simulink model "PV_WIND_BESS_ISLAND_R1"  (R2023b)
settings: Solver=ode14x  StartTime=0.0  StopTime=3.2  FixedStep=25e-6  MaxStep=1e-5  RelTol=1e-3
InitFcn:
  | setup_v2_paths;init_grid_supported_integration;run(which('init_bess_vsm_r10.m'));
undefined symbols (not defined in the file): Base, Control, Converter, DiscIntNeverNeededParam, Drive, Filter, G, PMSG, V2, Wind
libraries: nesl_utility x51, ee_lib x44, fl_lib x25, simulink x6
(part 2 of 4)

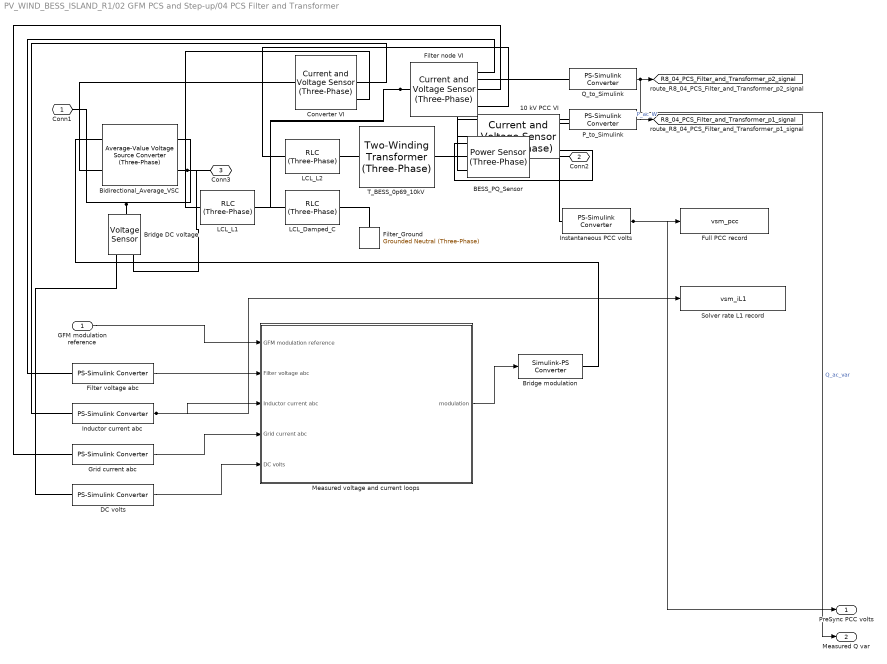
== system PV_WIND_BESS_ISLAND_R1/02 GFM PCS and Step-up/04 PCS Filter and Transformer ==
  GFM modulation reference : Inport
  10 kV PCC VI : ee_lib/Sensors & Transducers/Current and Voltage Sensor (Three-Phase)  port_option=ee.enum.threePhasePort.composite  vMeasurementType=ee.enum.vmeasurement.lg  outputUnit=ee.enum.unit.si  SRated=100e6 A*V  VRated=24e3 V  I_specify=off  I_priority=None  I=[0, 0, 0] A  I_nominal_specify=off  I_nominal_value=1  I_nominal_unit=A  V_specify=off  V_priority=None  V=[0, 0, 0] V  V_nominal_specify=off  V_nominal_value=1  V_nominal_unit=V
  BESS_PQ_Sensor : ee_lib/Sensors & Transducers/Power Sensor (Three-Phase)  port_option=ee.enum.threePhasePort.composite  load_type=ee.enum.passive.type_balanced.balanced  f0=60 Hz
  Bidirectional_Average_VSC : ee_lib/Semiconductors & Converters/Converters/Average-Value Voltage Source Converter (Three-Phase)  port_option=ee.enum.threePhasePort.composite  enable_block_pulses_input=false  krec=G.dc.Rbattery_ohm/10 Ohm  frequency_option=ee.enum.converters.frequency.variable  input_option=ee.enum.converters.inputOption.ModWave  FRated=G.f0_Hz Hz  losses_parameterization=ee.enum.converters.losses.fixed  Pfixed=1 W  ks=0.01  kc1=1.7 V  kc2=0.01 Ohm  Ploss_vect=[100, 800, 1870, 3250, 4900] W  Irms_vect=[10, 100, 200, 300, 400] A  Vdc_nom=300 V  thermal_mass=30000 J/K  temperature_specify=off  temperature_priority=High  temperature=298.15 K  temperature_nominal_specify=off  temperature_nominal_value=1  temperature_nominal_unit=K
  Bridge DC voltage : fl_lib/Electrical/Electrical Sensors/Voltage Sensor
  Bridge modulation : nesl_utility/Simulink-PS Converter  PhysicalDomain=network_engine_domain  SubClassName=ps_input  LeftPortType=input  RightPortType=output  PseudoPeriodic=off  Frequencies=[]  NoiseDistribution=none  NoiseParameters=[]  Unit=1  AffineConversion=off  FilteringAndDerivatives=zero  SimscapeFilterOrder=1  InputFilterTimeConstant=0.001  UdotUserProvided=0
  Converter VI : ee_lib/Sensors & Transducers/Current and Voltage Sensor (Three-Phase)  port_option=ee.enum.threePhasePort.composite  vMeasurementType=ee.enum.vmeasurement.lg  outputUnit=ee.enum.unit.si  SRated=100e6 A*V  VRated=24e3 V  I_specify=off  I_priority=None  I=[0, 0, 0] A  I_nominal_specify=off  I_nominal_value=1  I_nominal_unit=A  V_specify=off  V_priority=None  V=[0, 0, 0] V  V_nominal_specify=off  V_nominal_value=1  V_nominal_unit=V
  DC volts : nesl_utility/PS-Simulink Converter  PhysicalDomain=network_engine_domain  SubClassName=ps_output  LeftPortType=input  RightPortType=output  PseudoPeriodic=off  Frequencies=[]  VectorFormat=inherit  Unit=V  AffineConversion=off
  Filter node VI : ee_lib/Sensors & Transducers/Current and Voltage Sensor (Three-Phase)  port_option=ee.enum.threePhasePort.composite  vMeasurementType=ee.enum.vmeasurement.lg  outputUnit=ee.enum.unit.si  SRated=100e6 A*V  VRated=24e3 V  I_specify=off  I_priority=None  I=[0, 0, 0] A  I_nominal_specify=off  I_nominal_value=1  I_nominal_unit=A  V_specify=off  V_priority=None  V=[0, 0, 0] V  V_nominal_specify=off  V_nominal_value=1  V_nominal_unit=V
  Filter voltage abc : nesl_utility/PS-Simulink Converter  PhysicalDomain=network_engine_domain  SubClassName=ps_output  LeftPortType=input  RightPortType=output  PseudoPeriodic=off  Frequencies=[]  VectorFormat=inherit  Unit=V  AffineConversion=off
  Filter_Ground : ee_lib/Connectors & References/Grounded Neutral (Three-Phase)  port_option=ee.enum.threePhasePort.composite
  Full PCC record : ToWorkspace  VariableName=vsm_pcc  SaveFormat=Timeseries  SampleTime=-1
  Grid current abc : nesl_utility/PS-Simulink Converter  PhysicalDomain=network_engine_domain  SubClassName=ps_output  LeftPortType=input  RightPortType=output  PseudoPeriodic=off  Frequencies=[]  VectorFormat=inherit  Unit=A  AffineConversion=off
  Inductor current abc : nesl_utility/PS-Simulink Converter  PhysicalDomain=network_engine_domain  SubClassName=ps_output  LeftPortType=input  RightPortType=output  PseudoPeriodic=off  Frequencies=[]  VectorFormat=inherit  Unit=A  AffineConversion=off
  Instantaneous PCC volts : nesl_utility/PS-Simulink Converter  PhysicalDomain=network_engine_domain  SubClassName=ps_output  LeftPortType=input  RightPortType=output  PseudoPeriodic=off  Frequencies=[]  VectorFormat=inherit  Unit=V  AffineConversion=off
  LCL_Damped_C : ee_lib/Passive/RLC Assemblies/RLC (Three-Phase)  port_option=ee.enum.threePhasePort.composite  component_structure=ee.enum.rlc.structure.SeriesRC  R=G.filter.Rd_ohm Ohm  L=1e-3 H  C=G.filter.C_F F  R_parasitic=0 Ohm  G_parasitic=0 1/Ohm  IL_specify=off  IL_priority=High  IL=[0, 0, 0] A  IL_nominal_specify=off  IL_nominal_value=1  IL_nominal_unit=A  VC_specify=off  VC_priority=High  VC=[0, 0, 0] V  VC_nominal_specify=off  VC_nominal_value=1  VC_nominal_unit=V
  LCL_L1 : ee_lib/Passive/RLC Assemblies/RLC (Three-Phase)  port_option=ee.enum.threePhasePort.composite  component_structure=ee.enum.rlc.structure.SeriesRL  R=G.filter.R1_ohm Ohm  L=G.filter.L1_H H  C=1e-6 F  R_parasitic=0 Ohm  G_parasitic=0 1/Ohm  IL_specify=off  IL_priority=High  IL=[0, 0, 0] A  IL_nominal_specify=off  IL_nominal_value=1  IL_nominal_unit=A  VC_specify=off  VC_priority=High  VC=[0, 0, 0] V  VC_nominal_specify=off  VC_nominal_value=1  VC_nominal_unit=V
  LCL_L2 : ee_lib/Passive/RLC Assemblies/RLC (Three-Phase)  port_option=ee.enum.threePhasePort.composite  component_structure=ee.enum.rlc.structure.SeriesRL  R=G.filter.R2_ohm Ohm  L=G.filter.L2_H H  C=1e-6 F  R_parasitic=0 Ohm  G_parasitic=0 1/Ohm  IL_specify=off  IL_priority=High  IL=[0, 0, 0] A  IL_nominal_specify=off  IL_nominal_value=1  IL_nominal_unit=A  VC_specify=off  VC_priority=High  VC=[0, 0, 0] V  VC_nominal_specify=off  VC_nominal_value=1  VC_nominal_unit=V
  Measured voltage and current loops : Subsystem
  P_to_Simulink : nesl_utility/PS-Simulink Converter  PhysicalDomain=network_engine_domain  SubClassName=ps_output  LeftPortType=input  RightPortType=output  PseudoPeriodic=off  Frequencies=[]  VectorFormat=inherit  Unit=W  AffineConversion=off
  Q_to_Simulink : nesl_utility/PS-Simulink Converter  PhysicalDomain=network_engine_domain  SubClassName=ps_output  LeftPortType=input  RightPortType=output  PseudoPeriodic=off  Frequencies=[]  VectorFormat=inherit  Unit=W  AffineConversion=off
  Solver rate L1 record : ToWorkspace  VariableName=vsm_iL1  SaveFormat=Timeseries  SampleTime=-1
  T_BESS_0p69_10kV : ee_lib/Passive/Transformers/Two-Winding Transformer (Three-Phase)  SRated=G.transformer.S_VA A*V  FRated=G.f0_Hz Hz  Winding1Connection=ee.enum.windingconnection.delta1  VRated1=G.ac.Vll_low_V V  Winding2Connection=ee.enum.windingconnection.Yg  VRated2=G.ac.Vll_high_V V  CoreType=ee.enum.coretype.threelimb  pu_Rw1=G.transformer.pu_Rw1  pu_Rw2=G.transformer.pu_Rw2  leakage_reactance_option=ee.enum.transformer_leakage.include  pu_Xl1=G.transformer.pu_Xl1  pu_Xl2=G.transformer.pu_Xl2  magnetizing_resistance_option=ee.enum.transformer_magnetizingResistance.exclude  pu_Rm=500  magnetizing_reactance_option=ee.enum.transformer_magnetizingReactance.exclude  saturation_option=ee.enum.transformer_saturation.exclude  pu_Xm=500  current_data=[0, .002, 1, 2]  magnetic_flux_data=[0, 1.2, 1.5, 1.51]  pu_X0=0.5  i1_specify=off  i1_priority=None  i1=[0, 0, 0] A  i1_nominal_specify=off  i1_nominal_value=1  i1_nominal_unit=A  i2_specify=off  i2_priority=None  i2=[0, 0, 0] A  i2_nominal_specify=off  i2_nominal_value=1  i2_nominal_unit=A  phi_specify=off  phi_priority=None  phi=[0, 0, 0]  phi_nominal_specify=off  phi_nominal_value=1  phi_nominal_unit=1
  Conn1 : PMIOPort  Side=Right  ConnectionType=Connection: foundation.electrical.electrical
  Conn2 : PMIOPort  Port=2  Side=Right  ConnectionType=Connection: foundation.electrical.three_phase
  Conn3 : PMIOPort  Port=3  Side=Right  ConnectionType=Connection: foundation.electrical.electrical
  PreSync PCC volts : Outport
  Measured Q var : Outport  Port=2
  tag scope: R8_04_PCS_Filter_and_Transformer_p1_signal=global, R8_04_PCS_Filter_and_Transformer_p2_signal=global
  wires:
  P_to_Simulink/1 -> [R8_04_PCS_Filter_and_Transformer_p1_signal]  "P_ac_W"
  Q_to_Simulink/1 -> [R8_04_PCS_Filter_and_Transformer_p2_signal], Measured Q var/1  "Q_ac_var"
  GFM modulation reference/1 -> Measured voltage and current loops/1(GFM modulation reference)
  Filter voltage abc/1 -> Measured voltage and current loops/2(Filter voltage abc)
  Inductor current abc/1 -> Measured voltage and current loops/3(Inductor current abc), Solver rate L1 record/1
  Grid current abc/1 -> Measured voltage and current loops/4(Grid current abc)
  DC volts/1 -> Measured voltage and current loops/5(DC volts)
  Measured voltage and current loops/1(modulation) -> Bridge modulation/1
  Instantaneous PCC volts/1 -> Full PCC record/1, PreSync PCC volts/1
  connections:
  BESS_PQ_Sensor/RConn1 -- Conn2/RConn1
  BESS_PQ_Sensor/LConn3 -- Q_to_Simulink/LConn1
  LCL_Damped_C/RConn1 -- Filter_Ground/LConn1
  LCL_L2/RConn1 -- T_BESS_0p69_10kV/LConn1
  Conn3/RConn1 -- Bidirectional_Average_VSC/RConn2 -- Bridge DC voltage/RConn2
  BESS_PQ_Sensor/LConn2 -- P_to_Simulink/LConn1
  Bidirectional_Average_VSC/RConn1 -- Conn1/RConn1 -- Bridge DC voltage/LConn1
  Bidirectional_Average_VSC/LConn2 -- Converter VI/LConn1
  Converter VI/RConn3 -- LCL_L1/LConn1
  LCL_Damped_C/LConn1 -- LCL_L1/RConn1 -- Filter node VI/LConn1
  Filter node VI/RConn3 -- LCL_L2/LConn1
  Filter node VI/RConn1 -- Filter voltage abc/LConn1
  Converter VI/RConn2 -- Inductor current abc/LConn1
  Filter node VI/RConn2 -- Grid current abc/LConn1
  Bridge DC voltage/RConn1 -- DC volts/LConn1
  Bridge modulation/RConn1 -- Bidirectional_Average_VSC/LConn1
  T_BESS_0p69_10kV/RConn1 -- 10 kV PCC VI/LConn1
  10 kV PCC VI/RConn3 -- BESS_PQ_Sensor/LConn1
  10 kV PCC VI/RConn1 -- Instantaneous PCC volts/LConn1

== system PV_WIND_BESS_ISLAND_R1/PV Resource/01 PV Array ==
  Array VI : Mux  Inputs=2
  Current SI : nesl_utility/PS-Simulink Converter  PhysicalDomain=network_engine_domain  SubClassName=ps_output  LeftPortType=input  RightPortType=output  PseudoPeriodic=off  Frequencies=[]  VectorFormat=inherit  Unit=A  AffineConversion=off
  Irradiance : Constant  Value=V2.PV.dynamic.irradiance_Wpm2
  Irradiance PS : nesl_utility/Simulink-PS Converter  PhysicalDomain=network_engine_domain  SubClassName=ps_input  LeftPortType=input  RightPortType=output  PseudoPeriodic=off  Frequencies=[]  NoiseDistribution=none  NoiseParameters=[]  Unit=W/m^2  AffineConversion=off  FilteringAndDerivatives=zero  SimscapeFilterOrder=1  InputFilterTimeConstant=0.001  UdotUserProvided=0
  PV Array : ee_lib/Sources/Solar Cell  prm=1  Isc=V2.PV.dynamic.Isc_cell_A A  Voc=V2.PV.dynamic.Voc_cell_V V  Is=1e-6 A  Is2=0 A  Iph=7.34 A  Ir0=1000 W/m^2  ec=1.5  N2=2  Rs=0 Ohm  Rp=inf Ohm  N_series=V2.PV.dynamic.Nseries  N_parallel=V2.PV.dynamic.Nparallel  TIPH1=0 1/K  EG=1.11 eV  TXIS1=3  TXIS2=3  TRS1=0  TRP1=0  Tmeas=25 degC  TFIXED=V2.PV.dynamic.temperature_degC degC  thermal_mass=100 J/K  initial_temperature=25 degC
  PV Current : fl_lib/Electrical/Electrical Sensors/Current Sensor
  PV Input Capacitor : fl_lib/Electrical/Electrical Elements/Capacitor  c=V2.PV.dynamic.Cpv_F F  r=1e-6 Ohm  g=0 1/Ohm  i_specify=off  i_priority=None  i=0 A  i_nominal_specify=off  i_nominal_value=1  i_nominal_unit=A  v_specify=off  v_priority=None  v=0 V  v_nominal_specify=off  v_nominal_value=1  v_nominal_unit=V  vc_specify=on  vc_priority=High  vc=V2.PV.dynamic.Vmp_initial_V V  vc_nominal_specify=off  vc_nominal_value=1  vc_nominal_unit=V
  PV Voltage : fl_lib/Electrical/Electrical Sensors/Voltage Sensor
  Voltage SI : nesl_utility/PS-Simulink Converter  PhysicalDomain=network_engine_domain  SubClassName=ps_output  LeftPortType=input  RightPortType=output  PseudoPeriodic=off  Frequencies=[]  VectorFormat=inherit  Unit=V  AffineConversion=off
  arrayPlus : PMIOPort  Side=Right  ConnectionType=Connection: foundation.electrical.electrical
  arrayMinus : PMIOPort  Port=2  Side=Right  ConnectionType=Connection: foundation.electrical.electrical
  arrayVI : Outport
  wires:
  Array VI/1 -> arrayVI/1
  Current SI/1 -> Array VI/2
  Voltage SI/1 -> Array VI/1
  Irradiance/1 -> Irradiance PS/1
  connections:
  PV Current/RConn1 -- Current SI/LConn1
  PV Voltage/RConn1 -- Voltage SI/LConn1
  arrayMinus/RConn1 -- PV Input Capacitor/RConn1 -- PV Array/RConn1 -- PV Voltage/RConn2
  arrayPlus/RConn1 -- PV Voltage/LConn1 -- PV Current/RConn2 -- PV Input Capacitor/LConn1
  PV Array/LConn2 -- PV Current/LConn1
  Irradiance PS/RConn1 -- PV Array/LConn1

== system PV_WIND_BESS_ISLAND_R1/PV Resource/02 MPPT Boost and DC Link ==
  dispatch : Inport
  arrayVI : Inport  Port=2
  Array measurements : Demux  Outputs=2
  Average Boost : ee_lib/Semiconductors & Converters/Converters/Boost Converter  port_option=ee.enum.controlport.ps  device_type=ee.enum.converters.switchingdevice.averaged  Vf=0.8 V  Ron=0.001 Ohm  Rds=0.001 Ohm  Goff=1e-5 1/Ohm  Vgt=1 V  Vgt_off=-1 V  Ih=1 A  Vth=6 V  K=0  diode_param=ee.enum.converters.protectiondiode.nodynamics  diode_Vf=0.8 V  diode_Ron=0.001 Ohm  diode_Goff=1e-5 1/Ohm  diode_C=50 nF  diode_iRM=-235 A  diode_iF=300 A  diode_idot=-50 A/us  diode_trr_param=ee.enum.converters.diodetrr.trr_factor  diode_trr_factor=3  diode_trr=15 us  diode_Qrr=1500 s*uA  Lf=V2.PV.dynamic.Lboost_H H  Rl=V2.PV.dynamic.Rboost_ohm Ohm  Cf=1e-6 F  Rf=0.001 Ohm  snubber_type=ee.enum.converters.snubber.exclude  Cs=1e-7 F  Rs=0.1 Ohm  iL_specify=off  iL_priority=High  iL=0 A  iL_nominal_specify=off  iL_nominal_value=1  iL_nominal_unit=A  vc_specify=on  vc_priority=High  vc=V2.PV.dynamic.Vdc_ref_V V  vc_nominal_specify=off  vc_nominal_value=1  vc_nominal_unit=V
  Boost Current Record : ToWorkspace  VariableName=pv_boost_current  SaveFormat=Timeseries  SampleTime=-1
  Boost Current SI : nesl_utility/PS-Simulink Converter  PhysicalDomain=network_engine_domain  SubClassName=ps_output  LeftPortType=input  RightPortType=output  PseudoPeriodic=off  Frequencies=[]  VectorFormat=inherit  Unit=A  AffineConversion=off
  Boost Output Current : fl_lib/Electrical/Electrical Sensors/Current Sensor
  DC Ground : fl_lib/Electrical/Electrical Elements/Electrical Reference
  DC Link Capacitor : fl_lib/Electrical/Electrical Elements/Capacitor  c=V2.PV.dynamic.Cdc_F F  r=1e-6 Ohm  g=0 1/Ohm  i_specify=off  i_priority=None  i=0 A  i_nominal_specify=off  i_nominal_value=1  i_nominal_unit=A  v_specify=off  v_priority=None  v=0 V  v_nominal_specify=off  v_nominal_value=1  v_nominal_unit=V  vc_specify=on  vc_priority=High  vc=V2.PV.dynamic.Vdc_ref_V V  vc_nominal_specify=off  vc_nominal_value=1  vc_nominal_unit=V
  DC Link Voltage : fl_lib/Electrical/Electrical Sensors/Voltage Sensor
  DC Link Voltage SI : nesl_utility/PS-Simulink Converter  PhysicalDomain=network_engine_domain  SubClassName=ps_output  LeftPortType=input  RightPortType=output  PseudoPeriodic=off  Frequencies=[]  VectorFormat=inherit  Unit=V  AffineConversion=off
  Duty PS : nesl_utility/Simulink-PS Converter  PhysicalDomain=network_engine_domain  SubClassName=ps_input  LeftPortType=input  RightPortType=output  PseudoPeriodic=off  Frequencies=[]  NoiseDistribution=none  NoiseParameters=[]  Unit=1  AffineConversion=off  FilteringAndDerivatives=zero  SimscapeFilterOrder=1  InputFilterTimeConstant=0.001  UdotUserProvided=0
  Duty Sample Delay : UnitDelay  SampleTime=100e-6
  MPPT and Curtailment : Subsystem
  Telemetry Mux : Mux  Inputs=6
  arrayPlus : PMIOPort  Side=Left  ConnectionType=Connection: foundation.electrical.electrical
  arrayMinus : PMIOPort  Port=2  Side=Left  ConnectionType=Connection: foundation.electrical.electrical
  linkPlus : PMIOPort  Port=3  Side=Right  ConnectionType=Connection: foundation.electrical.electrical
  linkMinus : PMIOPort  Port=4  Side=Right  ConnectionType=Connection: foundation.electrical.electrical
  sourceData : Outport
  wires:
  Telemetry Mux/1 -> sourceData/1
  MPPT and Curtailment/3(Vpv_target) -> Telemetry Mux/6
  MPPT and Curtailment/2(Vmp) -> Telemetry Mux/5
  Duty Sample Delay/1 -> Duty PS/1
  MPPT and Curtailment/1(Duty) -> Telemetry Mux/4, Duty Sample Delay/1
  dispatch/1 -> MPPT and Curtailment/4(Command)
  DC Link Voltage SI/1 -> Telemetry Mux/3, MPPT and Curtailment/3(Vdc)
  Array measurements/2 -> Telemetry Mux/2, MPPT and Curtailment/2(Ipv)
  Array measurements/1 -> Telemetry Mux/1, MPPT and Curtailment/1(Vpv)
  arrayVI/1 -> Array measurements/1
  Boost Current SI/1 -> Boost Current Record/1
  connections:
  Duty PS/RConn1 -- Average Boost/LConn1
  DC Link Voltage/RConn1 -- DC Link Voltage SI/LConn1
  Boost Output Current/RConn1 -- Boost Current SI/LConn1
  linkMinus/RConn1 -- DC Link Capacitor/RConn1 -- DC Link Voltage/RConn2 -- DC Ground/LConn1 -- Average Boost/RConn2
  linkPlus/RConn1 -- DC Link Capacitor/LConn1 -- DC Link Voltage/LConn1 -- Boost Output Current/RConn2
  Average Boost/RConn1 -- Boost Output Current/LConn1
  arrayMinus/RConn1 -- Average Boost/LConn3
  arrayPlus/RConn1 -- Average Boost/LConn2

== system PV_WIND_BESS_ISLAND_R1/PV Resource/03 Average Grid Converter ==
  modulationABC : Inport
  Average VSC : ee_lib/Semiconductors & Converters/Converters/Average-Value Voltage Source Converter (Three-Phase)  port_option=ee.enum.threePhasePort.composite  enable_block_pulses_input=false  krec=0.01 Ohm  frequency_option=ee.enum.converters.frequency.variable  input_option=ee.enum.converters.inputOption.ModWave  FRated=V2.PV.rating.f_Hz Hz  losses_parameterization=ee.enum.converters.losses.fixed  Pfixed=1 W  ks=0.01  kc1=1.7 V  kc2=0.01 Ohm  Ploss_vect=[100, 800, 1870, 3250, 4900] W  Irms_vect=[10, 100, 200, 300, 400] A  Vdc_nom=V2.PV.dynamic.Vdc_ref_V V  thermal_mass=30000 J/K  temperature_specify=off  temperature_priority=High  temperature=298.15 K  temperature_nominal_specify=off  temperature_nominal_value=1  temperature_nominal_unit=K
  Converter VI : ee_lib/Sensors & Transducers/Current and Voltage Sensor (Three-Phase)  port_option=ee.enum.threePhasePort.composite  vMeasurementType=ee.enum.vmeasurement.lg  outputUnit=ee.enum.unit.si  SRated=100e6 A*V  VRated=24e3 V  I_specify=off  I_priority=None  I=[0, 0, 0] A  I_nominal_specify=off  I_nominal_value=1  I_nominal_unit=A  V_specify=off  V_priority=None  V=[0, 0, 0] V  V_nominal_specify=off  V_nominal_value=1  V_nominal_unit=V
  Converter Voltage Record : ToWorkspace  VariableName=pv_converter_vabc  SaveFormat=Timeseries  SampleTime=-1
  DC Current Record : ToWorkspace  VariableName=pv_vsc_dc_current  SaveFormat=Timeseries  SampleTime=-1
  DC Current SI : nesl_utility/PS-Simulink Converter  PhysicalDomain=network_engine_domain  SubClassName=ps_output  LeftPortType=input  RightPortType=output  PseudoPeriodic=off  Frequencies=[]  VectorFormat=inherit  Unit=A  AffineConversion=off
  Modulation PS : nesl_utility/Simulink-PS Converter  PhysicalDomain=network_engine_domain  SubClassName=ps_input  LeftPortType=input  RightPortType=output  PseudoPeriodic=off  Frequencies=[]  NoiseDistribution=none  NoiseParameters=[]  Unit=1  AffineConversion=off  FilteringAndDerivatives=zero  SimscapeFilterOrder=1  InputFilterTimeConstant=0.001  UdotUserProvided=0
  Modulation Sample Delay : UnitDelay  InitialCondition=[0;-0.39;0.39]  SampleTime=100e-6
  VSC DC Current : fl_lib/Electrical/Electrical Sensors/Current Sensor
  iabc SI : nesl_utility/PS-Simulink Converter  PhysicalDomain=network_engine_domain  SubClassName=ps_output  LeftPortType=input  RightPortType=output  PseudoPeriodic=off  Frequencies=[]  VectorFormat=inherit  Unit=A  AffineConversion=off
  vabc SI : nesl_utility/PS-Simulink Converter  PhysicalDomain=network_engine_domain  SubClassName=ps_output  LeftPortType=input  RightPortType=output  PseudoPeriodic=off  Frequencies=[]  VectorFormat=inherit  Unit=V  AffineConversion=off
  DC_Positive : PMIOPort  Side=Left  ConnectionType=Connection: foundation.electrical.electrical
  DC_Negative : PMIOPort  Port=2  Side=Left  ConnectionType=Connection: foundation.electrical.electrical
  AC_690V : PMIOPort  Port=3  Side=Right  ConnectionType=Connection: foundation.electrical.three_phase
  converterCurrentABC : Outport
  wires:
  iabc SI/1 -> converterCurrentABC/1
  Modulation Sample Delay/1 -> Modulation PS/1
  modulationABC/1 -> Modulation Sample Delay/1
  vabc SI/1 -> Converter Voltage Record/1
  DC Current SI/1 -> DC Current Record/1
  connections:
  Modulation PS/RConn1 -- Average VSC/LConn1
  Converter VI/RConn2 -- iabc SI/LConn1
  Converter VI/RConn1 -- vabc SI/LConn1
  Converter VI/RConn3 -- AC_690V/RConn1
  Average VSC/LConn2 -- Converter VI/LConn1
  DC_Negative/RConn1 -- Average VSC/RConn2
  VSC DC Current/RConn2 -- Average VSC/RConn1
  DC_Positive/RConn1 -- VSC DC Current/LConn1
  VSC DC Current/RConn1 -- DC Current SI/LConn1

== system PV_WIND_BESS_ISLAND_R1/PV Resource/04 Local GFL Control ==
  PCCMeasurementBus : Inport
  converterCurrentABC : Inport  Port=2
  sourceData : Inport  Port=3
  dispatch : Inport  Port=4
  01 Local PLL : Subsystem
      settings: AttributesFormatString=local PCC voltage only
  02 Measured dq : Subsystem
  03 Vdc and Q to current reference : Subsystem
  04 Current PI and voltage limit : Subsystem
  05 Voltage dq to modulation : Subsystem
  06 Control telemetry : Subsystem
  Grid Phase Voltage : Gain  Gain=[1 -1 0;0 1 -1;-1 0 1]*(V2.PV.rating.V_ac_low_V/V2.PV.rating.V_pcc_V)/3  Multiplication=Matrix(u*K)
  PCC Voltage : BusSelector  OutputSignals=vabc_V
  PCS Telemetry : Mux  Inputs=5
  Ppv : Fcn  Expr=u(1)*u(2)
  Vdc : Fcn  Expr=u(3)
  modulationABC : Outport
  controlData : Outport  Port=2
  wires:
  PCS Telemetry/1 -> controlData/1
  01 Local PLL/3(phase_error) -> PCS Telemetry/4
  01 Local PLL/2(omega) -> PCS Telemetry/3
  06 Control telemetry/1(Telemetry) -> PCS Telemetry/1
  05 Voltage dq to modulation/1(mabc) -> PCS Telemetry/5, modulationABC/1
  03 Vdc and Q to current reference/3(outer_status) -> 06 Control telemetry/3(outer_status)
  04 Current PI and voltage limit/1(voltage_dq) -> 05 Voltage dq to modulation/1(voltage_dq)
  03 Vdc and Q to current reference/2(enable) -> 04 Current PI and voltage limit/4(enable)
  03 Vdc and Q to current reference/1(reference_dq) -> 06 Control telemetry/1(reference_dq), 04 Current PI and voltage limit/2(reference_dq)
  dispatch/1 -> 03 Vdc and Q to current reference/4(Command)
  Ppv/1 -> 03 Vdc and Q to current reference/3(Ppv)
  Vdc/1 -> 05 Voltage dq to modulation/3(Vdc), 04 Current PI and voltage limit/3(Vdc), 03 Vdc and Q to current reference/2(Vdc)
  02 Measured dq/1(measured_dq) -> 06 Control telemetry/2(measured_dq), 04 Current PI and voltage limit/1(measured_dq), 03 Vdc and Q to current reference/1(measured_dq)
  01 Local PLL/1(theta) -> PCS Telemetry/2, 05 Voltage dq to modulation/2(theta), 02 Measured dq/3(theta)
  converterCurrentABC/1 -> 02 Measured dq/2(iabc)
  sourceData/1 -> Ppv/1, Vdc/1
  Grid Phase Voltage/1 -> 02 Measured dq/1(vabc), 01 Local PLL/1(Vabc)
  PCC Voltage/1 -> Grid Phase Voltage/1  "<vabc_V>"
  PCCMeasurementBus/1 -> PCC Voltage/1

== system PV_WIND_BESS_ISLAND_R1/PV Resource/05 Filter Transformer and PCC ==
  Damped Shunt C : ee_lib/Passive/RLC Assemblies/RLC (Three-Phase)  port_option=ee.enum.threePhasePort.composite  component_structure=ee.enum.rlc.structure.SeriesRC  R=V2.PV.filter.Rd_ohm Ohm  L=1e-3 H  C=V2.PV.filter.C_F F  R_parasitic=0 Ohm  G_parasitic=0 1/Ohm  IL_specify=off  IL_priority=High  IL=[0, 0, 0] A  IL_nominal_specify=off  IL_nominal_value=1  IL_nominal_unit=A  VC_specify=off  VC_priority=High  VC=[0, 0, 0] V  VC_nominal_specify=off  VC_nominal_value=1  VC_nominal_unit=V
  Filter Ground : ee_lib/Connectors & References/Grounded Neutral (Three-Phase)  port_option=ee.enum.threePhasePort.composite
  Grid-side R2 + L2 : ee_lib/Passive/RLC Assemblies/RLC (Three-Phase)  port_option=ee.enum.threePhasePort.composite  component_structure=ee.enum.rlc.structure.SeriesRL  R=V2.PV.filter.R2_ohm Ohm  L=V2.PV.filter.L2_H H  C=1e-6 F  R_parasitic=0 Ohm  G_parasitic=0 1/Ohm  IL_specify=off  IL_priority=High  IL=[0, 0, 0] A  IL_nominal_specify=off  IL_nominal_value=1  IL_nominal_unit=A  VC_specify=off  VC_priority=High  VC=[0, 0, 0] V  VC_nominal_specify=off  VC_nominal_value=1  VC_nominal_unit=V
  Inverter-side R1 + L1 : ee_lib/Passive/RLC Assemblies/RLC (Three-Phase)  port_option=ee.enum.threePhasePort.composite  component_structure=ee.enum.rlc.structure.SeriesRL  R=V2.PV.filter.R1_ohm Ohm  L=V2.PV.filter.L1_H H  C=1e-6 F  R_parasitic=0 Ohm  G_parasitic=0 1/Ohm  IL_specify=off  IL_priority=High  IL=[0, 0, 0] A  IL_nominal_specify=off  IL_nominal_value=1  IL_nominal_unit=A  VC_specify=off  VC_priority=High  VC=[0, 0, 0] V  VC_nominal_specify=off  VC_nominal_value=1  VC_nominal_unit=V
  PCC Measurement : Subsystem
  Step-up Transformer : ee_lib/Passive/Transformers/Two-Winding Transformer (Three-Phase)  SRated=V2.PV.transformer.S_VA A*V  FRated=V2.PV.rating.f_Hz Hz  Winding1Connection=ee.enum.windingconnection.Yg  VRated1=V2.PV.transformer.V1_V V  Winding2Connection=ee.enum.windingconnection.Yg  VRated2=V2.PV.transformer.V2_V V  CoreType=ee.enum.coretype.threelimb  pu_Rw1=V2.PV.transformer.R_pu/2  pu_Rw2=V2.PV.transformer.R_pu/2  leakage_reactance_option=ee.enum.transformer_leakage.exclude  pu_Xl1=0.05  pu_Xl2=0.05  magnetizing_resistance_option=ee.enum.transformer_magnetizingResistance.exclude  pu_Rm=500  magnetizing_reactance_option=ee.enum.transformer_magnetizingReactance.exclude  saturation_option=ee.enum.transformer_saturation.exclude  pu_Xm=500  current_data=[0, .002, 1, 2]  magnetic_flux_data=[0, 1.2, 1.5, 1.51]  pu_X0=0.5  i1_specify=off  i1_priority=None  i1=[0, 0, 0] A  i1_nominal_specify=off  i1_nominal_value=1  i1_nominal_unit=A  i2_specify=off  i2_priority=None  i2=[0, 0, 0] A  i2_nominal_specify=off  i2_nominal_value=1  i2_nominal_unit=A  phi_specify=off  phi_priority=None  phi=[0, 0, 0]  phi_nominal_specify=off  phi_nominal_value=1  phi_nominal_unit=1
  PCS AC Terminal : PMIOPort  Side=Left  ConnectionType=Connection: foundation.electrical.three_phase
  PCC_10kV : PMIOPort  Port=2  Side=Right  ConnectionType=Connection: foundation.electrical.three_phase
  PCCMeasurementBus : Outport  OutDataTypeStr=Bus: PCCMeasurementBus
  wires:
  PCC Measurement/1(PCCMeasurementBus) -> PCCMeasurementBus/1
  connections:
  PCC Measurement/RConn1 -- PCC_10kV/RConn1
  Step-up Transformer/RConn1 -- PCC Measurement/LConn1
  Grid-side R2 + L2/RConn1 -- Step-up Transformer/LConn1
  Damped Shunt C/RConn1 -- Filter Ground/LConn1
  Damped Shunt C/LConn1 -- Inverter-side R1 + L1/RConn1 -- Grid-side R2 + L2/LConn1
  PCS AC Terminal/RConn1 -- Inverter-side R1 + L1/LConn1

== system PV_WIND_BESS_ISLAND_R1/PV Resource/Command Interface ==
  Command : Inport
  Select gridDispatch : BusSelector  OutputSignals=Q_ref_var,enable  OutputAsBus=on
  Select mode : BusSelector  OutputSignals=mode
  Select sourceDispatch : BusSelector  OutputSignals=P_ref_W,enable  OutputAsBus=on
  sourceDispatch : Outport
  gridDispatch : Outport  Port=2
  mode : Outport  Port=3
  wires:
  Select mode/1 -> mode/1  "<mode>"
  Select gridDispatch/1 -> gridDispatch/1
  Select sourceDispatch/1 -> sourceDispatch/1
  Command/1 -> Select mode/1, Select gridDispatch/1, Select sourceDispatch/1

== system PV_WIND_BESS_ISLAND_R1/PV Resource/Resource Status ==
  PCC : Inport
  sourceData : Inport  Port=2
  controlData : Inport  Port=3
  mode : Inport  Port=4
  Commissioning recorder : Subsystem
  Current limit factor : Fcn  Expr=u(9)
  DC capability and health : Subsystem
  PCC values : BusSelector  OutputSignals=P_W,Q_var,Vll_rms_V
  PCC voltage alias : SignalConversion  OverrideOpt=off
  PLL frequency : Fcn  Expr=u(11)/(2*pi)
  Status fields : BusCreator  Inputs=11  OutDataTypeStr=Bus: ResourceStatusBus
  Status : Outport
  wires:
  Status fields/1 -> Status/1
  DC capability and health/5(outHealthy) -> Status fields/11  "healthy"
  mode/1 -> Status fields/10  "control_mode"
  DC capability and health/4(outVdc) -> Status fields/9  "Vdc_V"
  DC capability and health/3(outEnergy) -> Status fields/8  "energy_state_pu"
  Current limit factor/1 -> Status fields/7  "current_limit_factor"
  DC capability and health/2(outReserve) -> Status fields/6  "power_headroom_W"
  DC capability and health/1(outAvailable) -> Status fields/5  "available_power_W"
  PLL frequency/1 -> Status fields/4  "frequency_Hz"
  PCC voltage alias/1 -> Status fields/3  "Vpcc_V"
  PCC values/2 -> Status fields/2  "<Q_var>"
  PCC values/3 -> PCC voltage alias/1  "<Vll_rms_V>"
  controlData/1 -> Commissioning recorder/3(controlData), Current limit factor/1, PLL frequency/1
  sourceData/1 -> Commissioning recorder/2(sourceData), DC capability and health/2(sourceData)
  PCC values/1 -> Status fields/1, DC capability and health/1(measuredP)  "<P_W>"
  PCC/1 -> Commissioning recorder/1(PCC), PCC values/1

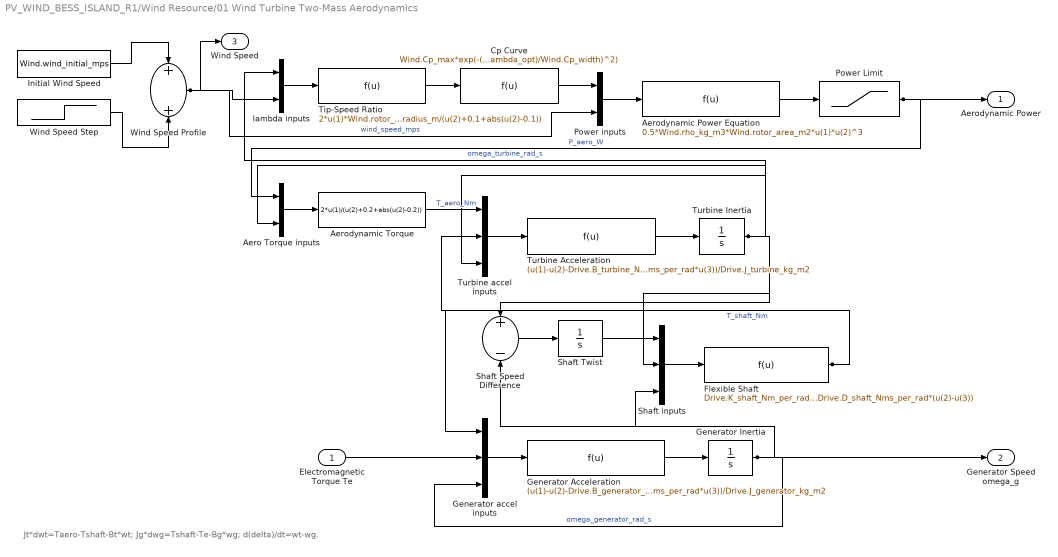
== system PV_WIND_BESS_ISLAND_R1/Wind Resource/01 Wind Turbine Two-Mass Aerodynamics ==
  note: Jt*dwt=Taero-Tshaft-Bt*wt; Jg*dwg=Tshaft-Te-Bg*wg; d(delta)/dt=wt-wg.
  Electromagnetic Torque Te : Inport
  Aero Torque inputs : Mux  Inputs=2
  Aerodynamic Power Equation : Fcn  Expr=0.5*Wind.rho_kg_m3*Wind.rotor_area_m2*u(1)*u(2)^3
  Aerodynamic Torque : Fcn  Expr=2*u(1)/(u(2)+0.2+abs(u(2)-0.2))
  Cp Curve : Fcn  Expr=Wind.Cp_max*exp(-((u-Wind.lambda_opt)/Wind.Cp_width)^2)
  Flexible Shaft : Fcn  Expr=Drive.K_shaft_Nm_per_rad*u(1)+Drive.D_shaft_Nms_per_rad*(u(2)-u(3))
  Generator Acceleration : Fcn  Expr=(u(1)-u(2)-Drive.B_generator_Nms_per_rad*u(3))/Drive.J_generator_kg_m2
  Generator Inertia : Integrator  InitialCondition=PMSG.Init.omega_rad_s
  Generator accel inputs : Mux  Inputs=3
  Initial Wind Speed : Constant  Value=Wind.wind_initial_mps
  Power Limit : Saturate  UpperLimit=1.10*Wind.P_rated_W  LowerLimit=0
  Power inputs : Mux  Inputs=2
  Shaft Speed Difference : Sum  Inputs=+-
  Shaft Twist : Integrator  InitialCondition=PMSG.Init.shaft_angle_rad
  Shaft inputs : Mux  Inputs=3
  Tip-Speed Ratio : Fcn  Expr=2*u(1)*Wind.rotor_radius_m/(u(2)+0.1+abs(u(2)-0.1))
  Turbine Acceleration : Fcn  Expr=(u(1)-u(2)-Drive.B_turbine_Nms_per_rad*u(3))/Drive.J_turbine_kg_m2
  Turbine Inertia : Integrator  InitialCondition=PMSG.Init.omega_rad_s
  Turbine accel inputs : Mux  Inputs=3
  Wind Speed Profile : Sum
  Wind Speed Step : Step  Time=10  After=Wind.wind_step_mps  SampleTime=0
  lambda inputs : Mux  Inputs=2
  Aerodynamic Power : Outport
  Generator Speed omega_g : Outport  Port=2
  Wind Speed : Outport  Port=3
  wires:
  Initial Wind Speed/1 -> Wind Speed Profile/1
  Wind Speed Step/1 -> Wind Speed Profile/2
  Wind Speed Profile/1 -> Wind Speed/1, lambda inputs/2, Power inputs/2  "wind_speed_mps"
  Turbine Inertia/1 -> lambda inputs/1, Aero Torque inputs/2, Turbine accel inputs/3, Shaft Speed Difference/1, Shaft inputs/2  "omega_turbine_rad_s"
  lambda inputs/1 -> Tip-Speed Ratio/1
  Tip-Speed Ratio/1 -> Cp Curve/1
  Cp Curve/1 -> Power inputs/1
  Power inputs/1 -> Aerodynamic Power Equation/1
  Aerodynamic Power Equation/1 -> Power Limit/1
  Power Limit/1 -> Aerodynamic Power/1, Aero Torque inputs/1  "P_aero_W"
  Aero Torque inputs/1 -> Aerodynamic Torque/1
  Aerodynamic Torque/1 -> Turbine accel inputs/1  "T_aero_Nm"
  Flexible Shaft/1 -> Turbine accel inputs/2, Generator accel inputs/1  "T_shaft_Nm"
  Turbine accel inputs/1 -> Turbine Acceleration/1
  Turbine Acceleration/1 -> Turbine Inertia/1
  Electromagnetic Torque Te/1 -> Generator accel inputs/2
  Generator Inertia/1 -> Generator accel inputs/3, Shaft Speed Difference/2, Shaft inputs/3, Generator Speed omega_g/1  "omega_generator_rad_s"
  Generator accel inputs/1 -> Generator Acceleration/1
  Generator Acceleration/1 -> Generator Inertia/1
  Shaft Speed Difference/1 -> Shaft Twist/1
  Shaft Twist/1 -> Shaft inputs/1
  Shaft inputs/1 -> Flexible Shaft/1

== system PV_WIND_BESS_ISLAND_R1/Wind Resource/02 PMSG dq Machine and Average MSC ==
  note: dq convention: generating iq < 0 and Te > 0. Voltage commands include cross-coupling and back-EMF feedforward plus circular Vdc limit.
  Generator Speed omega_g : Inport
  01 Torque and Current References : Subsystem
  02 MSC Current Control : Subsystem
  03 PMSG Electrical Dynamics : Subsystem
  04 MSC DC Power : Subsystem
  Electrical Speed : Gain  Gain=PMSG.pole_pairs
  Electromagnetic Torque Te : Outport
  MSC DC Power : Outport  Port=2
  wires:
  Generator Speed omega_g/1 -> Electrical Speed/1, 01 Torque and Current References/1(omega_g)
  01 Torque and Current References/1(id_ref) -> 02 MSC Current Control/1(id_ref)
  01 Torque and Current References/2(iq_ref) -> 02 MSC Current Control/2(iq_ref)
  Electrical Speed/1 -> 02 MSC Current Control/3(omega_e), 03 PMSG Electrical Dynamics/3(omega_e)
  03 PMSG Electrical Dynamics/2(id) -> 02 MSC Current Control/4(id), 04 MSC DC Power/3(id)
  03 PMSG Electrical Dynamics/3(iq) -> 02 MSC Current Control/5(iq), 04 MSC DC Power/4(iq)
  02 MSC Current Control/1(vd) -> 03 PMSG Electrical Dynamics/1(vd), 04 MSC DC Power/1(vd)
  02 MSC Current Control/2(vq) -> 03 PMSG Electrical Dynamics/2(vq), 04 MSC DC Power/2(vq)
  03 PMSG Electrical Dynamics/1(Te) -> Electromagnetic Torque Te/1
  04 MSC DC Power/1(Pdc) -> MSC DC Power/1

== system PV_WIND_BESS_ISLAND_R1/Wind Resource/03 DC Link and Two-Level GSC ==
  note: Physical path: precharge branch -> DC rail (Cdc, Vdc sensor and MSC current injection) -> two-level bridge -> AC measurement.
      | The MSC injects I=Pmsc/Vdc; the 1500 V support contactor opens at 100 ms, after which Cdc carries the energy mismatch.
  Pmsc : Inport
  Brake Current Monitor : Terminator
  Converter AC Measurement : Subsystem
  DC Control and Monitoring : Subsystem
  DC Negative Reference : fl_lib/Electrical/Electrical Elements/Electrical Reference
  DC Precharge Source : ee_lib/Sources/Voltage Source  dc_voltage=Converter.Vdc_nom V  ac_voltage=0 V  ac_shift=0 rad  ac_frequency=60 Hz  noise_mode=ee.enum.sources.noise.Disabled  PSD=0 V^2/Hz  sample_time=1e-3 s  repeatability=ee.enum.sources.repeatability.NotRepeatable  user_seed=0  auto_seed=3499211588  i_specify=off  i_priority=None  i=0 A  i_nominal_specify=off  i_nominal_value=1  i_nominal_unit=A  v_specify=off  v_priority=None  v=0 V  v_nominal_specify=off  v_nominal_value=1  v_nominal_unit=V
  DC-Link Capacitor : ee_lib/Passive/Capacitor  cap_option=ee.enum.passive.capacitor.capOption.const  c=Converter.Cdc F  Cvec=[1e-05, 1e-06] F  Vvec=[0, 10] V  CV_table_symmetry=ee.enum.passive.capacitor.tableSymmetry.yes  f_vec=[1, 10] kHz  DFext_vec=[.8, 1.2]  enable_C_tol=ee.enum.toleranceApplication.none  averaging_period=0 s  C_tol=5  tol_distribution=ee.enum.toleranceDistribution.uniform  nSigma=4  r=Converter.Cdc_esr Ohm  g=0 1/Ohm  enable_operating_limits=ee.enum.enable.no  operating_limit_action=ee.enum.passive.reportOpLim.warn  max_working_voltage_range=[-25, 25] V  power_rating=1 W  maxTemperature=85 degC  thermalEnable=false  thermalMass=1 J/K  i_specify=off  i_priority=None  i=0 A  i_nominal_specify=off  i_nominal_value=1  i_nominal_unit=A  v_specify=on  v_priority=High  v=Converter.Vdc_nom V  v_nominal_specify=off  v_nominal_value=1  v_nominal_unit=V  vc_specify=off  vc_priority=High  vc=0 V  vc_nominal_specify=off  vc_nominal_value=1  vc_nominal_unit=V  T_specify=off  T_priority=None  T=298.15 K  T_nominal_specify=off  T_nominal_value=1  T_nominal_unit=K
  MSC Current Injection : fl_lib/Electrical/Electrical Sources/Controlled Current Source
  MSC Current to Physical : nesl_utility/Simulink-PS Converter  PhysicalDomain=network_engine_domain  SubClassName=ps_input  LeftPortType=input  RightPortType=output  PseudoPeriodic=off  Frequencies=[]  NoiseDistribution=none  NoiseParameters=[]  Unit=A  AffineConversion=off  FilteringAndDerivatives=provide  SimscapeFilterOrder=1  InputFilterTimeConstant=0.001  UdotUserProvided=0
  Precharge Disconnect Switch : ee_lib/Semiconductors & Converters/Ideal Semiconductor Switch  port_option=ee.enum.controlport.ps  Ron=Wind.brake_switch_Ron_ohm Ohm  Goff=Wind.brake_switch_Goff_S 1/Ohm  Vth=0.5 V  diode_param=ee.enum.converters.protectiondiode.none  diode_Vf=0.8 V  diode_Ron=0.001 Ohm  diode_Goff=1e-5 1/Ohm  diode_C=50e-9 F  diode_iRM=-235 A  diode_iF=300 A  diode_idot=-50 A/us  diode_trr_param=ee.enum.converters.diodetrr.trr_factor  diode_trr_factor=3  diode_trr=15 us  diode_Qrr=1500 s*uA
  Precharge Gate to Physical : nesl_utility/Simulink-PS Converter  PhysicalDomain=network_engine_domain  SubClassName=ps_input  LeftPortType=input  RightPortType=output  PseudoPeriodic=off  Frequencies=[]  NoiseDistribution=none  NoiseParameters=[]  Unit=1  AffineConversion=off  FilteringAndDerivatives=provide  SimscapeFilterOrder=1  InputFilterTimeConstant=0.001  UdotUserProvided=0
  Precharge Open Command : Step  Time=Wind.precharge_open_time_s  Before=1  After=0  SampleTime=0
  Precharge Resistor : ee_lib/Passive/Resistor  R=Wind.precharge_R_ohm Ohm  enable_R_tol=ee.enum.toleranceApplication.none  R_tol=5  tol_distribution=ee.enum.toleranceDistribution.uniform  nSigma=4  enable_operating_limits=ee.enum.enable.no  operating_limit_action=ee.enum.passive.reportOpLim.warn  power_rating=1 W  max_working_voltage=100 V  noise_mode=ee.enum.sources.noise.Disabled  Tdevice=25 degC  sample_time=1e-3 s  repeatability=ee.enum.ic.repeatability.notRepeatable  user_seed=0  auto_seed=3890346746  power_derating_T1=70 degC  power_derating_T2=155 degC  operating_temperature_range_vec=[-50, 150] degC  alpha=3.93e-3 1/K  Tmeas=25 degC  thermal_mass=100 J/K  temperature_specify=off  temperature_priority=High  temperature=298.15 K  temperature_nominal_specify=off  temperature_nominal_value=1  temperature_nominal_unit=K
  Sampled Vdc Monitor : Terminator
  Two-Level Three-Phase Bridge : ee_lib/Semiconductors & Converters/Converters/Converter (Three-Phase)  port_option=ee.enum.threePhasePort.composite  fidelity_option=ee.enum.converters.fidelity.detailed  device_type=ee.enum.converters.switchingdevice.averaged  showThermalPort=false  K=0  Vth=Converter.GateThresholdVoltage V  Vgt=1 V  Vgt_off=-1 V  Ih=1 A  Vf=0.8 V  Ron=Converter.SwitchOnResistance Ohm  Rds=0.001 Ohm  Goff=Converter.OffConductance 1/Ohm  Eon_scalar=22.86e-3 J  Eoff_scalar=17.14e-3 J  Eoff_natural_commutation=10e-3 J  Voff=300 V  Iout_scalar=600 A  onCurrentMeasDelay=0 s  useCurrentFromPreviousCycle=false  useVoltageFromPreviousCycle=false  diode_param=ee.enum.converters.protectiondiode.nodynamics  diode_Vf=0.8 V  diode_Ron=0.001 Ohm  diode_Goff=1e-5 1/Ohm  diode_C=50 nF  diode_iRM=-235 A  diode_iF=300 A  diode_idot=-50 A/us  diode_trr_param=ee.enum.converters.diodetrr.trr_factor  diode_trr_factor=3  diode_trr=15 us  diode_Qrr=1500 s*uA  diode_rec_loss_model=ee.enum.diode.reverseRecoveryModel.fixed  diode_ErecVal=0 J  diode_scaleWithIandV=false  diode_ErecMat=zeros(2, 3) J  diode_TjrecVec=[298.15, 398.15] K  diode_IfrecVec=[.1, 1, 10] A  diode_IrecVal=10 A  diode_VrecVal=10 V  diode_tFilter=1 / 1000 / 100 s  thermal_network_parameterization=ee.enum.thermalNetworkTopology.external  Rth=[.08, .5] K/W  Rth_Cauer=[.08, .1, .5] K/W  Rth_Foster=[.08, .14, .22, .16] K/W  thermal_mass_parameterization=ee.enum.thermalNetwork.timeconstant  thermal_mass=[.01, .5] J/K  thermal_mass_Cauer=[.01, .1, .5] J/K  thermal_mass_Foster=[.001, .005, .05, .5] J/K  thermal_time_constant=[.001, .2] s  thermal_time_constant_Cauer=[.001, .1, .2] s  thermal_time_constant_Foster=[7e-05, .0007, .01, .08] s  thermal_mass_initial_temperatures=[25, 25] degC  thermal_mass_initial_temperatures_Cauer=[25, 25, 25] degC  junction_thermal_mass=0.01 J/K  Tvec_initial_Foster=[25, 25, 25, 25] degC  snubber_type=ee.enum.converters.snubber.exclude  Cs=1e-7 F  Rs=0.1 Ohm  Vce_loss=[0, 150, 300] V
  Vdc Sensor : fl_lib/Electrical/Electrical Sensors/Voltage Sensor
  Vdc to Simulink : nesl_utility/PS-Simulink Converter  PhysicalDomain=network_engine_domain  SubClassName=ps_output  LeftPortType=input  RightPortType=output  PseudoPeriodic=off  Frequencies=[]  VectorFormat=inherit  Unit=V  AffineConversion=off
  Gate Drive : PMIOPort  Side=Left
  AC_Terminal : PMIOPort  Port=2  Side=Right
  wires:
  Vdc to Simulink/1 -> DC Control and Monitoring/1(Vdc Measured)  "Vdc_Meas"
  Pmsc/1 -> DC Control and Monitoring/2(Pmsc)  "P_msc_W"
  DC Control and Monitoring/1(I_msc Command) -> MSC Current to Physical/1  "I_msc_A"
  DC Control and Monitoring/2(Sampled Vdc) -> Sampled Vdc Monitor/1  "Vdc_msc_sampled"
  DC Control and Monitoring/3(Brake Current) -> Brake Current Monitor/1  "brake_current_A"
  Precharge Open Command/1 -> Precharge Gate to Physical/1  "precharge_gate"
  connections:
  Gate Drive/RConn1 -- Two-Level Three-Phase Bridge/LConn1
  Vdc Sensor/RConn1 -- Vdc to Simulink/LConn1
  Two-Level Three-Phase Bridge/LConn2 -- Converter AC Measurement/LConn1
  Converter AC Measurement/RConn1 -- AC_Terminal/RConn1
  MSC Current to Physical/RConn1 -- MSC Current Injection/RConn1
  DC Precharge Source/LConn1 -- Precharge Disconnect Switch/RConn1
  Precharge Disconnect Switch/RConn2 -- Precharge Resistor/LConn1
  Vdc Sensor/LConn1 -- Precharge Resistor/RConn1 -- DC-Link Capacitor/LConn1 -- MSC Current Injection/LConn1 -- Two-Level Three-Phase Bridge/RConn1
  Vdc Sensor/RConn2 -- DC Precharge Source/RConn1 -- DC-Link Capacitor/RConn1 -- Two-Level Three-Phase Bridge/RConn2 -- MSC Current Injection/RConn2 -- DC Negative Reference/LConn1
  Precharge Gate to Physical/RConn1 -- Precharge Disconnect Switch/LConn1

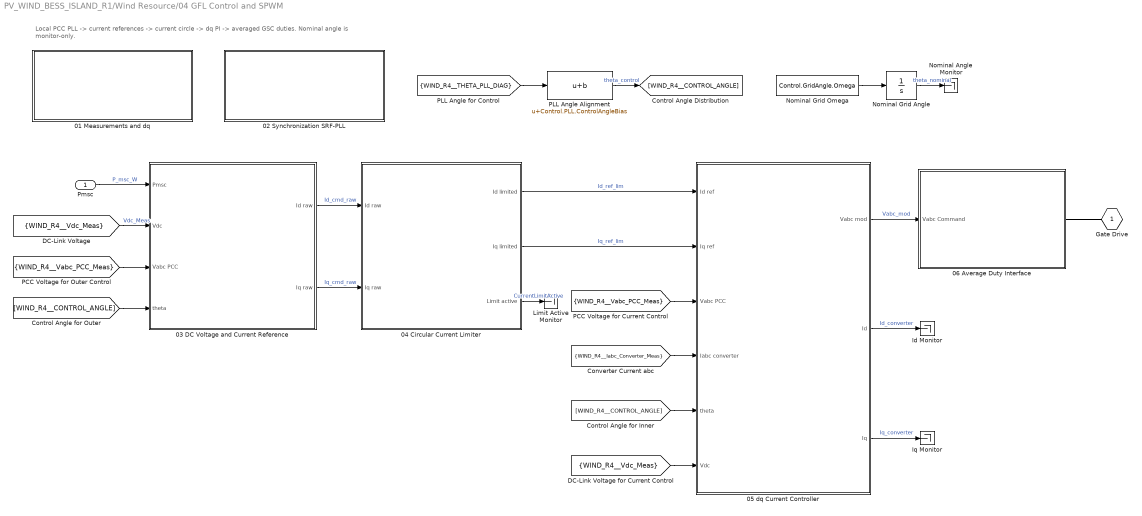
== system PV_WIND_BESS_ISLAND_R1/Wind Resource/04 GFL Control and SPWM ==
  note: Local PCC PLL -> current references -> current circle -> dq PI -> averaged GSC duties. Nominal angle is monitor-only.
  Pmsc : Inport
  01 Measurements and dq : Subsystem
  02 Synchronization SRF-PLL : Subsystem
  03 DC Voltage and Current Reference : Subsystem
  04 Circular Current Limiter : Subsystem
  05 dq Current Controller : Subsystem
  06 Average Duty Interface : Subsystem
  Id Monitor : Terminator
  Iq Monitor : Terminator
  Limit Active Monitor : Terminator
  Nominal Angle Monitor : Terminator
  Nominal Grid Angle : Integrator  InitialCondition=Control.GridAngle.Theta0
  Nominal Grid Omega : Constant  Value=Control.GridAngle.Omega
  PLL Angle Alignment : Bias  Bias=Control.PLL.ControlAngleBias  SaturateOnIntegerOverflow=off
  Gate Drive : PMIOPort  Side=Right
  wires:
  [WIND_R4__THETA_PLL_DIAG] -> PLL Angle Alignment/1
  05 dq Current Controller/1(Vabc mod) -> 06 Average Duty Interface/1(Vabc Command)  "Vabc_mod"
  Pmsc/1 -> 03 DC Voltage and Current Reference/1(Pmsc)  "P_msc_W"
  [WIND_R4__Vdc_Meas] -> 03 DC Voltage and Current Reference/2(Vdc)  "Vdc_Meas"
  [WIND_R4__Vabc_PCC_Meas] -> 03 DC Voltage and Current Reference/3(Vabc PCC)
  Nominal Grid Omega/1 -> Nominal Grid Angle/1
  PLL Angle Alignment/1 -> [WIND_R4__CONTROL_ANGLE]  "theta_control"
  [WIND_R4__CONTROL_ANGLE] -> 03 DC Voltage and Current Reference/4(theta)
  03 DC Voltage and Current Reference/1(Id raw) -> 04 Circular Current Limiter/1(Id raw)  "Id_cmd_raw"
  03 DC Voltage and Current Reference/2(Iq raw) -> 04 Circular Current Limiter/2(Iq raw)  "Iq_cmd_raw"
  04 Circular Current Limiter/1(Id limited) -> 05 dq Current Controller/1(Id ref)  "Id_ref_lim"
  04 Circular Current Limiter/2(Iq limited) -> 05 dq Current Controller/2(Iq ref)  "Iq_ref_lim"
  [WIND_R4__Vabc_PCC_Meas] -> 05 dq Current Controller/3(Vabc PCC)
  [WIND_R4__Iabc_Converter_Meas] -> 05 dq Current Controller/4(Iabc converter)
  [WIND_R4__CONTROL_ANGLE] -> 05 dq Current Controller/5(theta)
  [WIND_R4__Vdc_Meas] -> 05 dq Current Controller/6(Vdc)
  05 dq Current Controller/2(Id) -> Id Monitor/1  "Id_converter"
  05 dq Current Controller/3(Iq) -> Iq Monitor/1  "Iq_converter"
  04 Circular Current Limiter/3(Limit active) -> Limit Active Monitor/1  "CurrentLimitActive"
  Nominal Grid Angle/1 -> Nominal Angle Monitor/1  "theta_nominal"
  connections:
  06 Average Duty Interface/RConn1 -- Gate Drive/RConn1

== system PV_WIND_BESS_ISLAND_R1/Wind Resource/05 Filter Transformer and PCC ==
  note: Direct power path: Rf + Lf -> 0.69/10 kV Y-Y transformer -> PCC VI sensor. Measurements remain internal and logged.
  0.69 kV to 10 kV Step-Up Transformer : ee_lib/Passive/Transformers/Two-Winding Transformer (Three-Phase)  SRated=Transformer.Sn A*V  FRated=Transformer.f Hz  Winding1Connection=ee.enum.windingconnection.Y  VRated1=Transformer.Vll_primary V  Winding2Connection=ee.enum.windingconnection.Y  VRated2=Transformer.Vll_secondary V  CoreType=ee.enum.coretype.threelimb  pu_Rw1=Transformer.R1_pu  pu_Rw2=Transformer.R2_pu  leakage_reactance_option=ee.enum.transformer_leakage.exclude  pu_Xl1=Transformer.X1_pu  pu_Xl2=Transformer.X2_pu  magnetizing_resistance_option=ee.enum.transformer_magnetizingResistance.exclude  pu_Rm=500  magnetizing_reactance_option=ee.enum.transformer_magnetizingReactance.exclude  saturation_option=ee.enum.transformer_saturation.exclude  pu_Xm=Transformer.Xm_pu  current_data=[0, .002, 1, 2]  magnetic_flux_data=[0, 1.2, 1.5, 1.51]  pu_X0=0.5  i1_specify=off  i1_priority=None  i1=[0, 0, 0] A  i1_nominal_specify=off  i1_nominal_value=1  i1_nominal_unit=A  i2_specify=off  i2_priority=None  i2=[0, 0, 0] A  i2_nominal_specify=off  i2_nominal_value=1  i2_nominal_unit=A  phi_specify=off  phi_priority=None  phi=[0, 0, 0]  phi_nominal_specify=off  phi_nominal_value=1  phi_nominal_unit=1
  AC Filter Rf + Lf : ee_lib/Passive/RLC Assemblies/RLC (Three-Phase)  port_option=ee.enum.threePhasePort.composite  component_structure=ee.enum.rlc.structure.SeriesRL  R=Filter.R Ohm  L=Filter.L H  C=1e-6 F  R_parasitic=0 Ohm  G_parasitic=0 1/Ohm  IL_specify=off  IL_priority=High  IL=[0, 0, 0] A  IL_nominal_specify=off  IL_nominal_value=1  IL_nominal_unit=A  VC_specify=off  VC_priority=High  VC=[0, 0, 0] V  VC_nominal_specify=off  VC_nominal_value=1  VC_nominal_unit=V
  Iabc PCC to Simulink : nesl_utility/PS-Simulink Converter  PhysicalDomain=network_engine_domain  SubClassName=ps_output  LeftPortType=input  RightPortType=output  PseudoPeriodic=off  Frequencies=[]  VectorFormat=inherit  Unit=A  AffineConversion=off
  PCC VI Sensor : ee_lib/Sensors & Transducers/Current and Voltage Sensor (Three-Phase)  port_option=ee.enum.threePhasePort.composite  vMeasurementType=ee.enum.vmeasurement.lg  outputUnit=ee.enum.unit.si  SRated=Base.Sn A*V  VRated=Base.Vll_hv V  I_specify=off  I_priority=None  I=[0, 0, 0] A  I_nominal_specify=off  I_nominal_value=1  I_nominal_unit=A  V_specify=off  V_priority=None  V=[0, 0, 0] V  V_nominal_specify=off  V_nominal_value=1  V_nominal_unit=V
  Vabc PCC to Simulink : nesl_utility/PS-Simulink Converter  PhysicalDomain=network_engine_domain  SubClassName=ps_output  LeftPortType=input  RightPortType=output  PseudoPeriodic=off  Frequencies=[]  VectorFormat=inherit  Unit=V  AffineConversion=off
  From_VSC : PMIOPort  Side=Left
  To_Grid : PMIOPort  Port=2  Side=Right
  tag scope: WIND_R4__Iabc_PCC_Meas=scoped, WIND_R4__Vabc_PCC_Meas=scoped
  wires:
  Vabc PCC to Simulink/1 -> [WIND_R4__Vabc_PCC_Meas]  "Vabc_PCC_Meas"
  Iabc PCC to Simulink/1 -> [WIND_R4__Iabc_PCC_Meas]  "Iabc_PCC_Meas"
  connections:
  From_VSC/RConn1 -- AC Filter Rf + Lf/LConn1
  AC Filter Rf + Lf/RConn1 -- 0.69 kV to 10 kV Step-Up Transformer/LConn1
  0.69 kV to 10 kV Step-Up Transformer/RConn1 -- PCC VI Sensor/LConn1
  PCC VI Sensor/RConn3 -- To_Grid/RConn1
  PCC VI Sensor/RConn1 -- Vabc PCC to Simulink/LConn1
  PCC VI Sensor/RConn2 -- Iabc PCC to Simulink/LConn1

== system PV_WIND_BESS_ISLAND_R1/Wind Resource/Command Interface ==
  ResourceCommandBus : Inport  OutDataTypeStr=Bus: ResourceCommandBus
  Command Selector : BusSelector  OutputSignals=P_ref_W,Q_ref_var,enable
  tag scope: WIND_R4__DISPATCH_W=scoped, WIND_R4__ENABLE=scoped, WIND_R4__Q_REF_VAR=scoped
  wires:
  Command Selector/3 -> [WIND_R4__ENABLE]  "<enable>"
  Command Selector/2 -> [WIND_R4__Q_REF_VAR]  "<Q_ref_var>"
  Command Selector/1 -> [WIND_R4__DISPATCH_W]  "<P_ref_W>"
  ResourceCommandBus/1 -> Command Selector/1
